simulink model "Vienna_Rectifier_PQ_Control"  (R2023b)
settings: Solver=VariableStepAuto  StartTime=0.0  StopTime=0.4  RelTol=1e-3
libraries: spsSeriesRLCBranchLib x6, spsIGBTLib x6, spsIGBTDiodeLib x6, spsVoltageMeasurementLib x5, spsCurrentMeasurementLib x3, spsRMSLib x3, spsACVoltageSourceLib x3, spsMeanLib x2, slpidlib x1, spsTHDLib x1, simulink x1, spspowerguiLib x1
settings Model: SimulationMode=accelerator  Creator=LXS  LastModifiedBy=Qu
settings SolverCC: ZeroCrossAlgorithm=Adaptive

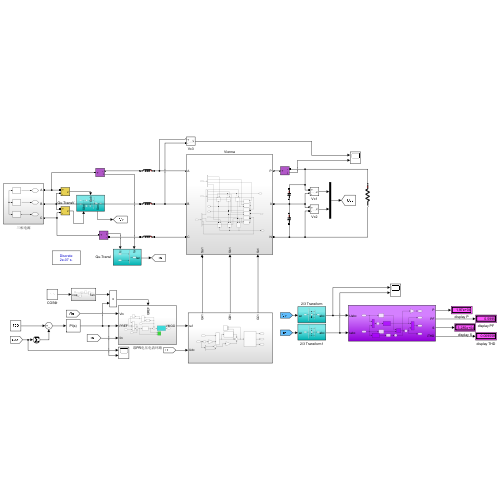
[thumbnail: Simulink's stored preview of the top-level diagram]
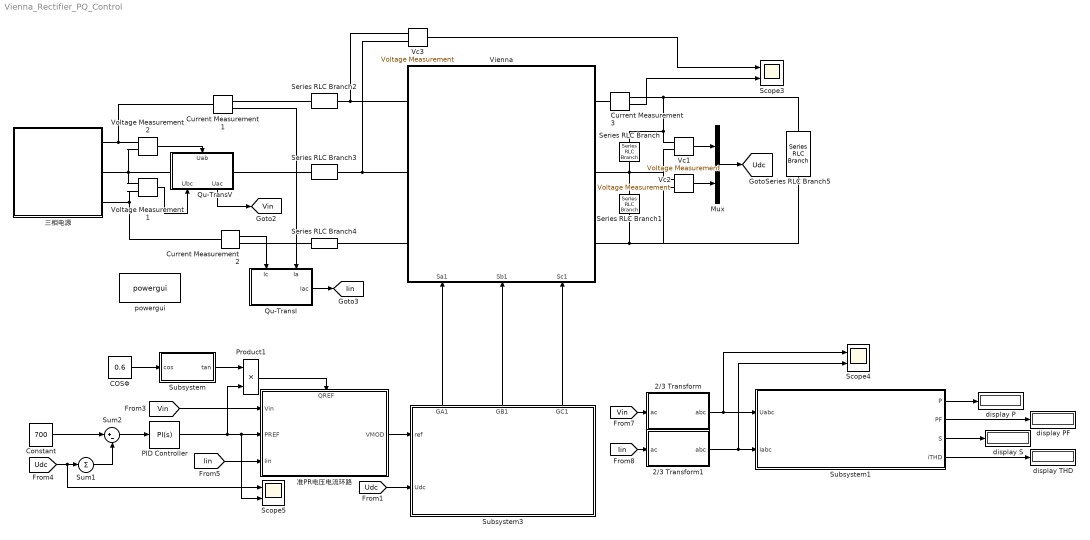
== system Vienna_Rectifier_PQ_Control ==
  2/3 Transform : Subsystem
      settings: PortSchema="{\"entries\":[{\"content\":{\"sides\":[{\"content\":{},\"type\":\"ConnectorPlacement.EquallySpacedRectSide\",\"uuid\":\"58c40194-9a95-4e39-952e-f878bde7484e\"},{\"content\":{\"side\":\"RIGHT\"},\"type\":\"ConnectorPlacement.EquallySpacedRectSide\",\"uuid\":\"f51692e8-3ff2-4d72-808d-3667196a4526\"},{\"content\":{\"connectorIds\":[\"In1\"],\"side\":\"TOP\"},\"type\":\"ConnectorPlacement.EquallySpacedRectSide\",\"uuid\":\"0aab136b-5da5-45c4-8998-999ebe8b7f2f\"},{\"content\":{\"connectorIds\":[\"Out1\"],\"side\":\"BOTTOM\"},\"type\":\"ConnectorPlacement.EquallySpacedRectSide\",\"uuid\":\"32f5f4a5-4ebb-496b-828d-b973bd46b44e\"}]},\"type\":\"ConnectorPlacement.EquallySpacedConnector\",\"uuid\":\"3ef81af7-d426-47fb-88e3-e33e58eebb83\"}],\"packageUris\":[\"http://schema.mathworks.com/mf0/Connector/R2020b\"],\"version\":\"1.0\"}"
  2/3 Transform1 : Subsystem
      settings: PortSchema="{\"entries\":[{\"content\":{\"sides\":[{\"content\":{},\"type\":\"ConnectorPlacement.EquallySpacedRectSide\",\"uuid\":\"58c40194-9a95-4e39-952e-f878bde7484e\"},{\"content\":{\"side\":\"RIGHT\"},\"type\":\"ConnectorPlacement.EquallySpacedRectSide\",\"uuid\":\"f51692e8-3ff2-4d72-808d-3667196a4526\"},{\"content\":{\"connectorIds\":[\"In1\"],\"side\":\"TOP\"},\"type\":\"ConnectorPlacement.EquallySpacedRectSide\",\"uuid\":\"0aab136b-5da5-45c4-8998-999ebe8b7f2f\"},{\"content\":{\"connectorIds\":[\"Out1\"],\"side\":\"BOTTOM\"},\"type\":\"ConnectorPlacement.EquallySpacedRectSide\",\"uuid\":\"32f5f4a5-4ebb-496b-828d-b973bd46b44e\"}]},\"type\":\"ConnectorPlacement.EquallySpacedConnector\",\"uuid\":\"3ef81af7-d426-47fb-88e3-e33e58eebb83\"}],\"packageUris\":[\"http://schema.mathworks.com/mf0/Connector/R2020b\"],\"version\":\"1.0\"}"
  COSΦ : Constant  Value=0.6
  Constant : Constant  Value=700
  Current Measurement1 : spsCurrentMeasurementLib/Current Measurement  PhasorSimulation=off  OutputType=Complex  PSBequivalent=0
  Current Measurement2 : spsCurrentMeasurementLib/Current Measurement  PhasorSimulation=off  OutputType=Complex  PSBequivalent=0
  Current Measurement3 : spsCurrentMeasurementLib/Current Measurement  PhasorSimulation=off  OutputType=Complex  PSBequivalent=0
  Mux : Mux  Inputs=2
  PID Controller : slpidlib/PID Controller  Controller=PI  Form=Parallel  TimeDomain=Continuous-time  UseExternalTs=off  SampleTime=-1  IntegratorMethod=Forward Euler  FilterMethod=Forward Euler  ControllerParametersSource=internal  P=0.15  I=10  UseKiTs=off  D=0  N=100  UseFilter=on  TunerSelectOption=Transfer Function Based (PID Tuner App)  InitialConditionSource=internal  InitialConditionForIntegrator=0  InitialConditionForFilter=0  DifferentiatorICPrevScaledInput=0  ExternalReset=none  TrackingMode=off  Kt=1  LimitOutput=off  SatLimitsSource=internal  UpperSaturationLimit=100  LowerSaturationLimit=-100  LinearizeAsGain=on  AntiWindupMode=none  Kb=1  LimitIntegrator=off  UpperIntegratorSaturationLimit=inf  LowerIntegratorSaturationLimit=-inf  POutMin=[]  POutMax=[]  IOutMin=[]  IOutMax=[]  DOutMin=[]  DOutMax=[]  NOutMin=[]  NOutMax=[]  SumOutMin=[]  SumOutMax=[]  SaturationOutMin=[]  SaturationOutMax=[]  PParamMin=[]  PParamMax=[]  IParamMin=[]  IParamMax=[]  DParamMin=[]  DParamMax=[]  NParamMin=[]  NParamMax=[]  KbParamMin=[]  KbParamMax=[]  KtParamMin=[]  KtParamMax=[]  KbOutMin=[]  KbOutMax=[]  KtOutMin=[]  KtOutMax=[]  IntegratorOutMin=[]  IntegratorOutMax=[]  FilterOutMin=[]  FilterOutMax=[]  SumI1OutMin=[]  SumI1OutMax=[]  SumI2OutMin=[]  SumI2OutMax=[]  SumI3OutMin=[]  SumI3OutMax=[]  SumI4OutMin=[]  SumI4OutMax=[]  SumDOutMin=[]  SumDOutMax=[]  DifferentiatorOutMin=[]  DifferentiatorOutMax=[]  FilterDiffOutCoefMin=[]  FilterDiffOutCoefMax=[]  ReciprocalOutMin=[]  ReciprocalOutMax=[]  SumDenOutMin=[]  SumDenOutMax=[]  SumNumOutMin=[]  SumNumOutMax=[]  DivideOutMin=[]  DivideOutMax=[]  UdiffTsProdOutMin=[]  UdiffTsProdOutMax=[]  NTsProdOutMin=[]  NTsProdOutMax=[]  UintegralTsProdOutMin=[]  UintegralTsProdOutMax=[]  UngainTsProdOutMin=[]  UngainTsProdOutMax=[]  ClampingZeroOutDataTypeStr=Inherit: Inherit via back propagation  ClampingZeroOutMin=[]  ClampingZeroOutMax=[]  FilterDenConstantOutDataTypeStr=Inherit: Inherit via back propagation  FilterDenConstantOutMin=[]  FilterDenConstantOutMax=[]  PCopyOutDataTypeStr=Inherit: Inherit via back propagation  PCopyOutMin=[]  PCopyOutMax=[]  NCopyOutDataTypeStr=Inherit: Inherit via back propagation  NCopyOutMin=[]  NCopyOutMax=[]  IntegratorContinuousStateAttributes=''  IntegratorStateMustResolveToSignalObject=off  IntegratorRTWStateStorageClass=Auto  FilterContinuousStateAttributes=''  FilterStateMustResolveToSignalObject=off  FilterRTWStateStorageClass=Auto  ParallelPVariant=InternalParameters  IdealPVariant=Disabled  IVariant=InternalParameters  DVariant=Disabled  IntegratorVariant=Continuous  SatVariant=Disabled  AWVariant=Passthrough  PCopyVariant=Disabled  TRVariant=Disabled  FdbkBlocksVariant=Forward  IdealPFdbkVariant=Disabled  SatFdbkVariant=Disabled  DerivativeFilterVariant=Disabled  NVariant=Disabled  NCopyVariant=Disabled_SignalSpec  FilterICVariant=Disabled  IntegratorICVariant=InternalICs  ExternalResetVariant=Disabled  TRSumVariant=Passthrough  SumFdbkVariant=Disabled  SumVariant=Sum_PI  TsampFilterVariant=InternalTs  TsampNgainVariant=Passthrough  TsampIntegralVariant=Disabled_SignalSpec  ExternalSaturationOutDataTypeStr=Inherit: Same as second input
  Product1 : Product
  Qu-TransI : Subsystem
      settings: PortSchema="{\"entries\":[{\"content\":{\"sides\":[{\"content\":{\"connectorIds\":[\"In1\",\"In2\"]},\"type\":\"ConnectorPlacement.EquallySpacedRectSide\",\"uuid\":\"58c40194-9a95-4e39-952e-f878bde7484e\"},{\"content\":{\"connectorIds\":[],\"side\":\"RIGHT\"},\"type\":\"ConnectorPlacement.EquallySpacedRectSide\",\"uuid\":\"f51692e8-3ff2-4d72-808d-3667196a4526\"},{\"content\":{\"connectorIds\":[],\"side\":\"TOP\"},\"type\":\"ConnectorPlacement.EquallySpacedRectSide\",\"uuid\":\"0aab136b-5da5-45c4-8998-999ebe8b7f2f\"},{\"content\":{\"connectorIds\":[\"Out1\"],\"side\":\"BOTTOM\"},\"type\":\"ConnectorPlacement.EquallySpacedRectSide\",\"uuid\":\"32f5f4a5-4ebb-496b-828d-b973bd46b44e\"}]},\"type\":\"ConnectorPlacement.EquallySpacedConnector\",\"uuid\":\"3ef81af7-d426-47fb-88e3-e33e58eebb83\"}],\"packageUris\":[\"http://schema.mathworks.com/mf0/Connector/R2020b\"],\"version\":\"1.0\"}"
  Qu-TransV : Subsystem
      settings: PortSchema="{\"entries\":[{\"content\":{\"sides\":[{\"content\":{\"connectorIds\":[\"In1\"]},\"type\":\"ConnectorPlacement.EquallySpacedRectSide\",\"uuid\":\"58c40194-9a95-4e39-952e-f878bde7484e\"},{\"content\":{\"connectorIds\":[\"In2\",\"Out1\"],\"side\":\"RIGHT\"},\"type\":\"ConnectorPlacement.EquallySpacedRectSide\",\"uuid\":\"f51692e8-3ff2-4d72-808d-3667196a4526\"},{\"content\":{\"side\":\"TOP\"},\"type\":\"ConnectorPlacement.EquallySpacedRectSide\",\"uuid\":\"0aab136b-5da5-45c4-8998-999ebe8b7f2f\"},{\"content\":{\"side\":\"BOTTOM\"},\"type\":\"ConnectorPlacement.EquallySpacedRectSide\",\"uuid\":\"185ce796-68e2-4136-8080-97dc86d2ba54\"}]},\"type\":\"ConnectorPlacement.EquallySpacedConnector\",\"uuid\":\"3ef81af7-d426-47fb-88e3-e33e58eebb83\"}],\"packageUris\":[\"http://schema.mathworks.com/mf0/Connector/R2020b\"],\"version\":\"1.0\"}"
  Scope3 : Scope  NumInputPorts=2
  Scope4 : Scope  NumInputPorts=2
  Scope5 : Scope  NumInputPorts=2
  Series RLC Branch : spsSeriesRLCBranchLib/Series RLC Branch  LConnTagsString=__new0  RConnTagsString=__new0  BranchType=C  Resistance=1  Inductance=1e-3  SetiL0=off  InitialCurrent=0  Capacitance=2e-3  Setx0=on  InitialVoltage=300  Measurements=None
  Series RLC Branch1 : spsSeriesRLCBranchLib/Series RLC Branch  LConnTagsString=__new0  RConnTagsString=__new0  BranchType=C  Resistance=1  Inductance=1e-3  SetiL0=off  InitialCurrent=0  Capacitance=2e-3  Setx0=on  InitialVoltage=300  Measurements=None
  Series RLC Branch2 : spsSeriesRLCBranchLib/Series RLC Branch  LConnTagsString=__new0  RConnTagsString=__new0  BranchType=L  Resistance=1  Inductance=5e-4  SetiL0=off  InitialCurrent=0  Capacitance=1e-6  Setx0=off  InitialVoltage=0  Measurements=None
  Series RLC Branch3 : spsSeriesRLCBranchLib/Series RLC Branch  LConnTagsString=__new0  RConnTagsString=__new0  BranchType=L  Resistance=1  Inductance=5e-4  SetiL0=off  InitialCurrent=0  Capacitance=1e-6  Setx0=off  InitialVoltage=0  Measurements=None
  Series RLC Branch4 : spsSeriesRLCBranchLib/Series RLC Branch  LConnTagsString=__new0  RConnTagsString=__new0  BranchType=L  Resistance=1  Inductance=5e-4  SetiL0=off  InitialCurrent=0  Capacitance=1e-6  Setx0=off  InitialVoltage=0  Measurements=None
  Series RLC Branch5 : spsSeriesRLCBranchLib/Series RLC Branch  LConnTagsString=__new0  RConnTagsString=__new0  BranchType=R  Resistance=25  Inductance=1e-3  SetiL0=off  InitialCurrent=0  Capacitance=1e-6  Setx0=off  InitialVoltage=0  Measurements=None
  Subsystem : Subsystem
  Subsystem1 : Subsystem
  Subsystem3 : Subsystem
      settings: PortSchema="{\"entries\":[{\"content\":{\"sides\":[{\"content\":{\"connectorIds\":[\"In1\",\"In2\"]},\"type\":\"ConnectorPlacement.EquallySpacedRectSide\",\"uuid\":\"86d8a801-af54-4615-919a-9a70996995f5\"},{\"content\":{\"side\":\"RIGHT\"},\"type\":\"ConnectorPlacement.EquallySpacedRectSide\",\"uuid\":\"9c099dd5-197a-4a29-8cd5-6822de601230\"},{\"content\":{\"connectorIds\":[\"Out1\",\"Out2\",\"Out3\"],\"side\":\"TOP\"},\"type\":\"ConnectorPlacement.EquallySpacedRectSide\",\"uuid\":\"5852d946-2383-4602-be71-32d16fa24bc3\"}]},\"type\":\"ConnectorPlacement.EquallySpacedConnector\",\"uuid\":\"a21c857f-e780-49b2-9a65-1676cf4540b1\"}],\"packageUris\":[\"http://schema.mathworks.com/mf0/Connector/R2020b\"],\"version\":\"1.0\"}"
  Sum1 : Sum  Inputs=+
  Sum2 : Sum  Inputs=|+-
  Vc1 : spsVoltageMeasurementLib/Voltage Measurement  PhasorSimulation=off  OutputType=Complex  PSBequivalent=0
  Vc2 : spsVoltageMeasurementLib/Voltage Measurement  PhasorSimulation=off  OutputType=Complex  PSBequivalent=0
  Vc3 : spsVoltageMeasurementLib/Voltage Measurement  PhasorSimulation=off  OutputType=Complex  PSBequivalent=0
  Vienna : Subsystem
      settings: PortSchema="{\"entries\":[{\"content\":{\"sides\":[{\"content\":{\"connectorIds\":[\"LConn1\",\"LConn2\",\"LConn3\"]},\"type\":\"ConnectorPlacement.EquallySpacedRectSide\",\"uuid\":\"b14efc91-6835-4ed7-8c1d-e2670cf7c179\"},{\"content\":{\"connectorIds\":[\"RConn1\",\"RConn2\",\"RConn3\"],\"side\":\"RIGHT\"},\"type\":\"ConnectorPlacement.EquallySpacedRectSide\",\"uuid\":\"133f26b8-b252-4d3c-80df-0b09760e0c14\"},{\"content\":{\"side\":\"TOP\"},\"type\":\"ConnectorPlacement.EquallySpacedRectSide\",\"uuid\":\"c058e102-7791-48c2-b9e4-e80cedcfd34e\"},{\"content\":{\"connectorIds\":[\"In1\",\"In2\",\"In3\"],\"side\":\"BOTTOM\"},\"type\":\"ConnectorPlacement.EquallySpacedRectSide\",\"uuid\":\"7bcd8845-3331-4b31-8039-611891643c20\"}]},\"type\":\"ConnectorPlacement.EquallySpacedConnector\",\"uuid\":\"173e4324-58a1-473c-9df3-d0606e4a673f\"}],\"packageUris\":[\"http://schema.mathworks.com/mf0/Connector/R2020b\"],\"version\":\"1.0\"}"
  Voltage Measurement1 : spsVoltageMeasurementLib/Voltage Measurement  PhasorSimulation=off  OutputType=Complex  PSBequivalent=0
  Voltage Measurement2 : spsVoltageMeasurementLib/Voltage Measurement  PhasorSimulation=off  OutputType=Complex  PSBequivalent=0
  display P : Display
  display PF : Display
  display S : Display
  display THD : Display
  powergui : spspowerguiLib/powergui  Priority=1  SimulationMode=Discrete  SampleTime=2e-7  frequency=60  Iterations=50  frequencyindice=50  Pbase=100e6  ErrMax=1e-4  UnitsV=kV  UnitsW=MW  buscounter=0  FunctionMessages=off  echomessages=off  EnableUseOfTLC=off  CurrentSourceSwitches=off  DisableSnubberDevices=off  DisableRonSwitches=off  DisableVfSwitches=off  DisplayEquations=off  AutomaticDiscreteSolvers=off  SolverType=Tustin/Backward Euler (TBE)  Interpol=off  ExternalGateDelay=off  methode=off  Ts=100  x0status=blocks  SPID=on  SwTol=0  HookPort=off  NonlinearTolerance=1e-4  nMaxIteration=100  ContinueOnMaxIteration=off  RestoreLinks=warning  ResistiveCurrentMeasurement=off  Frange=[0:2:500]  Ylog=off  Xlog=on  ShowGrid=off  save=off  variable=ZData  structure=0  ZoomFFT=off  StartTime=0.0  cycles=1  DisplayStyle=1  fundamental=60  FreqAxis=off  MaxFrequency=1000  frequencyindicesteady=1  RmsSteady=1  display=off
  三相电源 : Subsystem
  准PR电压电流环路 : Subsystem
      settings: PortSchema="{\"entries\":[{\"content\":{\"sides\":[{\"content\":{\"connectorIds\":[\"In1\",\"In2\",\"In3\"]},\"type\":\"ConnectorPlacement.EquallySpacedRectSide\",\"uuid\":\"dac3ff54-d1de-481a-901d-fe7d7474e460\"},{\"content\":{\"connectorIds\":[\"Out1\"],\"side\":\"RIGHT\"},\"type\":\"ConnectorPlacement.EquallySpacedRectSide\",\"uuid\":\"94b949b8-63b3-457c-8ea5-da44edec9bf3\"},{\"content\":{\"connectorIds\":[\"In4\"],\"side\":\"TOP\"},\"type\":\"ConnectorPlacement.EquallySpacedRectSide\",\"uuid\":\"1f5417c1-0a8c-48b6-bea3-1dc4e853aed2\"}]},\"type\":\"ConnectorPlacement.EquallySpacedConnector\",\"uuid\":\"5b0aae56-5e7d-4c0c-ad53-99d1136af505\"}],\"packageUris\":[\"http://schema.mathworks.com/mf0/Connector/R2020b\"],\"version\":\"1.0\"}"
  tag scope: Iin=global, Udc=global, Vin=global
  wires:
  Vc1/1 -> Mux/1
  Vc2/1 -> Mux/2
  Constant/1 -> Sum2/1
  Sum1/1 -> Sum2/2
  Sum2/1 -> PID Controller/1
  [Vin] -> 准PR电压电流环路/1(Vin)
  [Udc] -> Subsystem3/2(Udc)
  Subsystem1/3(S) -> display S/1
  Subsystem1/4(iTHD) -> display THD/1
  Subsystem1/2(PF) -> display PF/1
  Subsystem1/1(P) -> display P/1
  Subsystem3/3(GC1) -> Vienna/3(Sc1)
  Subsystem3/1(GA1) -> Vienna/1(Sa1)
  Subsystem3/2(GB1) -> Vienna/2(Sb1)
  [Udc] -> Scope5/1, Sum1/1
  Mux/1 -> [Udc]
  Vc3/1 -> Scope3/1
  Voltage Measurement2/1 -> Qu-TransV/1(Uab)
  Voltage Measurement1/1 -> Qu-TransV/2(Ubc)
  Qu-TransV/1(Uac) -> [Vin]
  Current Measurement2/1 -> Qu-TransI/1(Ic)
  Current Measurement1/1 -> Qu-TransI/2(Ia)
  Qu-TransI/1(Iac) -> [Iin]
  准PR电压电流环路/1(VMOD) -> Subsystem3/1(ref)
  PID Controller/1 -> Product1/2, Scope5/2, 准PR电压电流环路/2(PREF)
  [Iin] -> 准PR电压电流环路/3(Iin)
  2/3 Transform1/1(abc) -> Subsystem1/2(Iabc), Scope4/2
  2/3 Transform/1(abc) -> Subsystem1/1(Uabc), Scope4/1
  [Iin] -> 2/3 Transform1/1(ac)
  [Vin] -> 2/3 Transform/1(ac)
  Current Measurement3/1 -> Scope3/2
  Product1/1 -> 准PR电压电流环路/4(QREF)
  Subsystem/1(tan) -> Product1/1
  COSΦ/1 -> Subsystem/1(cos)
  connections:
  Series RLC Branch2/LConn1 -- Vienna/LConn1 -- Vc3/LConn1
  Series RLC Branch3/LConn1 -- Vc3/LConn2 -- Vienna/LConn2
  Series RLC Branch4/LConn1 -- Vienna/LConn3
  Series RLC Branch/RConn1 -- Vc1/LConn2 -- Vc2/LConn1 -- Series RLC Branch1/LConn1 -- Vienna/RConn2
  Series RLC Branch5/LConn1 -- Vc1/LConn1 -- Series RLC Branch/LConn1 -- Current Measurement3/RConn1
  三相电源/RConn1 -- Voltage Measurement2/LConn1 -- Current Measurement1/LConn1
  三相电源/RConn2 -- Voltage Measurement2/LConn2 -- Voltage Measurement1/LConn1 -- Series RLC Branch3/RConn1
  三相电源/RConn3 -- Current Measurement2/LConn1 -- Voltage Measurement1/LConn2
  Current Measurement1/RConn1 -- Series RLC Branch2/RConn1
  Current Measurement2/RConn1 -- Series RLC Branch4/RConn1
  Series RLC Branch1/RConn1 -- Series RLC Branch5/RConn1 -- Vc2/LConn2 -- Vienna/RConn3
  Current Measurement3/LConn1 -- Vienna/RConn1

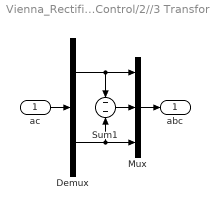
== system Vienna_Rectifier_PQ_Control/2//3 Transform ==
  ac : Inport
  Demux : Demux  Outputs=2
  Mux : Mux  Inputs=3
  Sum1 : Sum  Inputs=-|-
  abc : Outport
  wires:
  Sum1/1 -> Mux/2
  Mux/1 -> abc/1
  Demux/1 -> Sum1/1, Mux/1
  ac/1 -> Demux/1
  Demux/2 -> Sum1/2, Mux/3

== system Vienna_Rectifier_PQ_Control/2//3 Transform1 ==
  ac : Inport
  Demux : Demux  Outputs=2
  Mux : Mux  Inputs=3
  Sum1 : Sum  Inputs=-|-
  abc : Outport
  wires:
  Sum1/1 -> Mux/2
  Mux/1 -> abc/1
  Demux/1 -> Sum1/1, Mux/1
  ac/1 -> Demux/1
  Demux/2 -> Sum1/2, Mux/3

== system Vienna_Rectifier_PQ_Control/Qu-TransI ==
  Ic : Inport
  Ia : Inport  Port=2
  Mux : Mux  Inputs=2
  Iac : Outport
  wires:
  Ia/1 -> Mux/1
  Mux/1 -> Iac/1
  Ic/1 -> Mux/2

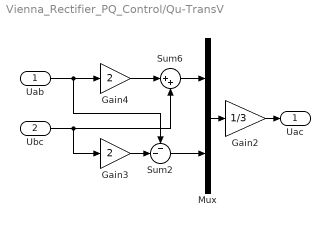
== system Vienna_Rectifier_PQ_Control/Qu-TransV ==
  Uab : Inport
  Ubc : Inport  Port=2
  Gain2 : Gain  Gain=1/3
  Gain3 : Gain  Gain=2
  Gain4 : Gain  Gain=2
  Mux : Mux  Inputs=2
  Sum2 : Sum  Inputs=--|
  Sum6 : Sum  Inputs=|++
  Uac : Outport
  wires:
  Uab/1 -> Sum2/1, Gain4/1
  Gain4/1 -> Sum6/1
  Ubc/1 -> Gain3/1, Sum6/2
  Sum2/1 -> Mux/2
  Sum6/1 -> Mux/1
  Gain3/1 -> Sum2/2
  Mux/1 -> Gain2/1
  Gain2/1 -> Uac/1

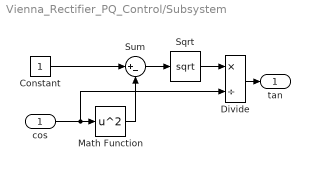
== system Vienna_Rectifier_PQ_Control/Subsystem ==
  cos : Inport
  Constant : Constant
  Divide : Product  Inputs=*/
  Math Function : Math  Operator=square
  Sqrt : Sqrt
  Sum : Sum  Inputs=|+-
  tan : Outport
  wires:
  cos/1 -> Divide/2, Math Function/1
  Math Function/1 -> Sum/2
  Constant/1 -> Sum/1
  Sum/1 -> Sqrt/1
  Sqrt/1 -> Divide/1
  Divide/1 -> tan/1

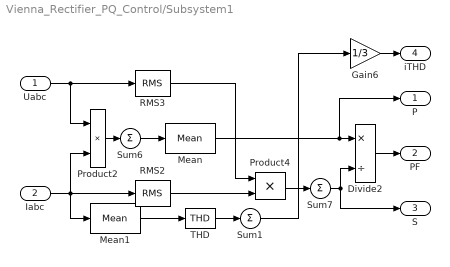
== system Vienna_Rectifier_PQ_Control/Subsystem1 ==
  Uabc : Inport
  Iabc : Inport  Port=2
  Divide2 : Product  Inputs=*/
  Gain6 : Gain  Gain=1/3
  Mean : spsMeanLib/Mean  Freq=100  Vinit=0  Ts=0
  Mean1 : spsMeanLib/Mean  Freq=20000  Vinit=0  Ts=0
  Product2 : Product
  Product4 : Product
  RMS2 : spsRMSLib/RMS  TrueRMS=on  Freq=50  RMSInit=0  Ts=0
  RMS3 : spsRMSLib/RMS  TrueRMS=on  Freq=50  RMSInit=0  Ts=0
  Sum1 : Sum  Inputs=+
  Sum6 : Sum  Inputs=+
  Sum7 : Sum  Inputs=+
  THD : spsTHDLib/THD  Freq=50  Ts=0
  P : Outport
  PF : Outport  Port=2
  S : Outport  Port=3
  iTHD : Outport  Port=4
  wires:
  Mean1/1 -> THD/1
  THD/1 -> Sum1/1
  Iabc/1 -> RMS2/1, Product2/2, Mean1/1
  Mean/1 -> Divide2/1, P/1
  Sum7/1 -> Divide2/2, S/1
  Uabc/1 -> Product2/1, RMS3/1
  Gain6/1 -> iTHD/1
  Sum1/1 -> Gain6/1
  RMS2/1 -> Product4/2
  Divide2/1 -> PF/1
  Product2/1 -> Sum6/1
  Sum6/1 -> Mean/1
  Product4/1 -> Sum7/1
  RMS3/1 -> Product4/1

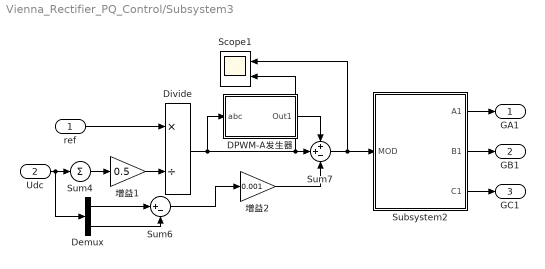
== system Vienna_Rectifier_PQ_Control/Subsystem3 ==
  ref : Inport
  Udc : Inport  Port=2
  DPWM-A发生器 : Subsystem
  Demux : Demux  Outputs=2
  Divide : Product  Inputs=*/
  Scope1 : Scope  NumInputPorts=2
  Subsystem2 : Subsystem
  Sum4 : Sum  Inputs=+
  Sum6 : Sum  Inputs=|+-
  Sum7 : Sum  Inputs=++-
  增益1 : Gain  Gain=0.5
  增益2 : Gain  Gain=0.001
  GA1 : Outport
  GB1 : Outport  Port=2
  GC1 : Outport  Port=3
  wires:
  Udc/1 -> Demux/1, Sum4/1
  ref/1 -> Divide/1
  Divide/1 -> Scope1/2, Sum7/2, DPWM-A发生器/1(abc)
  Sum7/1 -> Subsystem2/1(MOD), Scope1/1
  增益1/1 -> Divide/2
  Sum4/1 -> 增益1/1
  Subsystem2/3(C1) -> GC1/1
  Subsystem2/2(B1) -> GB1/1
  Subsystem2/1(A1) -> GA1/1
  DPWM-A发生器/1(Out1) -> Sum7/1
  Demux/1 -> Sum6/1
  Demux/2 -> Sum6/2
  Sum6/1 -> 增益2/1
  增益2/1 -> Sum7/3

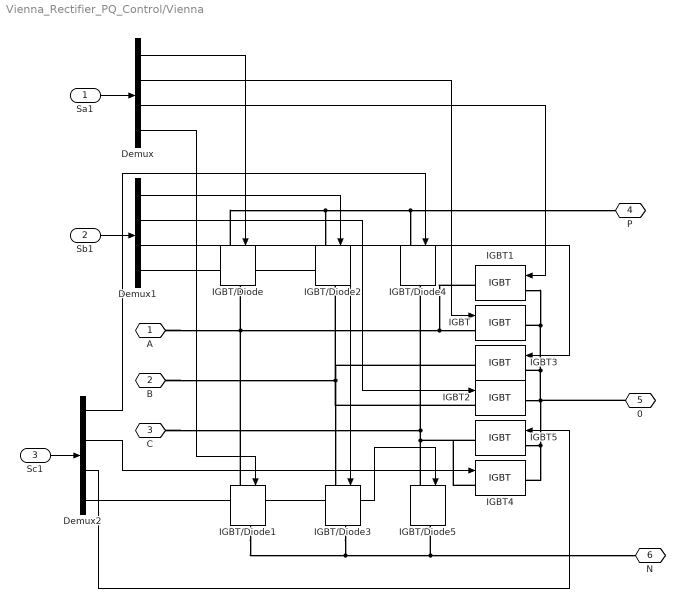
== system Vienna_Rectifier_PQ_Control/Vienna ==
  Sa1 : Inport
  Sb1 : Inport  Port=2
  Sc1 : Inport  Port=3
  Demux : Demux
  Demux1 : Demux
  Demux2 : Demux
  IGBT{,1..5} (6 alike) : spsIGBTLib/IGBT  Ron=0.001  Lon=0  Vf=1  Tf=1e-6  Tt=2e-6  IC=0  Rs=1e5  Cs=inf  Measurements=off
  IGBT/Diode{,1..5} (6 alike) : spsIGBTDiodeLib/IGBT//Diode  Ron=1e-3  Rs=1e5  Cs=inf  Measurements=off
  A : PMIOPort  Side=Left
  B : PMIOPort  Port=2  Side=Left
  C : PMIOPort  Port=3  Side=Left
  P : PMIOPort  Port=4  Side=Right
  0 : PMIOPort  Port=5  Side=Right
  N : PMIOPort  Port=6  Side=Right
  wires:
  Sa1/1 -> Demux/1
  Sb1/1 -> Demux1/1
  Sc1/1 -> Demux2/1
  Demux/2 -> IGBT/1
  Demux/3 -> IGBT1/1
  Demux/4 -> IGBT/Diode1/1
  Demux1/2 -> IGBT2/1
  Demux1/3 -> IGBT3/1
  Demux1/4 -> IGBT/Diode3/1
  Demux2/1 -> IGBT/Diode4/1
  Demux2/3 -> IGBT5/1
  Demux2/4 -> IGBT/Diode5/1
  Demux/1 -> IGBT/Diode/1
  Demux1/1 -> IGBT/Diode2/1
  Demux2/2 -> IGBT4/1
  connections:
  C/RConn1 -- IGBT4/LConn1 -- IGBT5/RConn1 -- IGBT/Diode5/LConn1 -- IGBT/Diode4/RConn1
  B/RConn1 -- IGBT2/LConn1 -- IGBT/Diode3/LConn1 -- IGBT/Diode2/RConn1 -- IGBT3/RConn1
  A/RConn1 -- IGBT/Diode/RConn1 -- IGBT1/RConn1 -- IGBT/LConn1 -- IGBT/Diode1/LConn1
  IGBT/Diode1/RConn1 -- IGBT/Diode3/RConn1 -- N/RConn1 -- IGBT/Diode5/RConn1
  IGBT/Diode/LConn1 -- IGBT/Diode2/LConn1 -- IGBT/Diode4/LConn1 -- P/RConn1
  IGBT2/RConn1 -- 0/RConn1 -- IGBT/RConn1 -- IGBT1/LConn1 -- IGBT3/LConn1 -- IGBT4/RConn1 -- IGBT5/LConn1

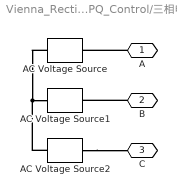
== system Vienna_Rectifier_PQ_Control/三相电源 ==
  AC Voltage Source : spsACVoltageSourceLib/AC Voltage Source  Amplitude=310  Phase=0  Frequency=50  SampleTime=0  Measurements=None  BusType=swing  Pref=10e3  Qref=0  Qmin=-inf  Qmax=+inf
  AC Voltage Source1 : spsACVoltageSourceLib/AC Voltage Source  Amplitude=310  Phase=120  Frequency=50  SampleTime=0  Measurements=None  BusType=swing  Pref=10e3  Qref=0  Qmin=-inf  Qmax=+inf
  AC Voltage Source2 : spsACVoltageSourceLib/AC Voltage Source  Amplitude=310  Phase=-120  Frequency=50  SampleTime=0  Measurements=None  BusType=swing  Pref=10e3  Qref=0  Qmin=-inf  Qmax=+inf
  A : PMIOPort  Side=Right
  B : PMIOPort  Port=2  Side=Right
  C : PMIOPort  Port=3  Side=Right
  connections:
  AC Voltage Source2/RConn1 -- C/RConn1
  A/RConn1 -- AC Voltage Source/RConn1
  B/RConn1 -- AC Voltage Source1/RConn1
  AC Voltage Source/LConn1 -- AC Voltage Source2/LConn1 -- AC Voltage Source1/LConn1

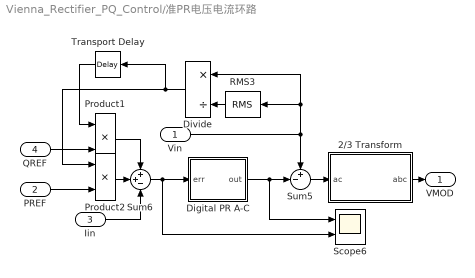
== system Vienna_Rectifier_PQ_Control/准PR电压电流环路 ==
  Vin : Inport
  PREF : Inport  Port=2
  Iin : Inport  Port=3
  QREF : Inport  Port=4
  2/3 Transform : Subsystem
      settings: PortSchema="{\"entries\":[{\"content\":{\"sides\":[{\"content\":{},\"type\":\"ConnectorPlacement.EquallySpacedRectSide\",\"uuid\":\"58c40194-9a95-4e39-952e-f878bde7484e\"},{\"content\":{\"side\":\"RIGHT\"},\"type\":\"ConnectorPlacement.EquallySpacedRectSide\",\"uuid\":\"f51692e8-3ff2-4d72-808d-3667196a4526\"},{\"content\":{\"connectorIds\":[\"In1\"],\"side\":\"TOP\"},\"type\":\"ConnectorPlacement.EquallySpacedRectSide\",\"uuid\":\"0aab136b-5da5-45c4-8998-999ebe8b7f2f\"},{\"content\":{\"connectorIds\":[\"Out1\"],\"side\":\"BOTTOM\"},\"type\":\"ConnectorPlacement.EquallySpacedRectSide\",\"uuid\":\"32f5f4a5-4ebb-496b-828d-b973bd46b44e\"}]},\"type\":\"ConnectorPlacement.EquallySpacedConnector\",\"uuid\":\"3ef81af7-d426-47fb-88e3-e33e58eebb83\"}],\"packageUris\":[\"http://schema.mathworks.com/mf0/Connector/R2020b\"],\"version\":\"1.0\"}"
  Digital PR A-C : Subsystem  mask{Kp=8, Kr=100, Wc=5, Ts=1/40000, Upper=600, Lower=-600}
      mask DialogControl ParameterGroupVar Prompt: 参数
  Divide : Product  Inputs=*/
  Product1 : Product
  Product2 : Product
  RMS3 : spsRMSLib/RMS  TrueRMS=on  Freq=50  RMSInit=220  Ts=0
  Scope6 : Scope  NumInputPorts=2
  Sum5 : Sum  Inputs=+-|
  Sum6 : Sum  Inputs=++-
  Transport Delay : TransportDelay  DelayTime=1/50/4
  VMOD : Outport
  wires:
  PREF/1 -> Product2/2
  Sum6/1 -> Digital PR A-C/1(err), Scope6/2
  Digital PR A-C/1(out) -> Scope6/1, Sum5/2
  Sum5/1 -> 2/3 Transform/1(ac)
  2/3 Transform/1(abc) -> VMOD/1
  Vin/1 -> Sum5/1, Divide/1, RMS3/1
  Iin/1 -> Sum6/3
  Product2/1 -> Sum6/2
  Product1/1 -> Sum6/1
  QREF/1 -> Product1/2
  RMS3/1 -> Divide/2
  Divide/1 -> Transport Delay/1, Product2/1
  Transport Delay/1 -> Product1/1

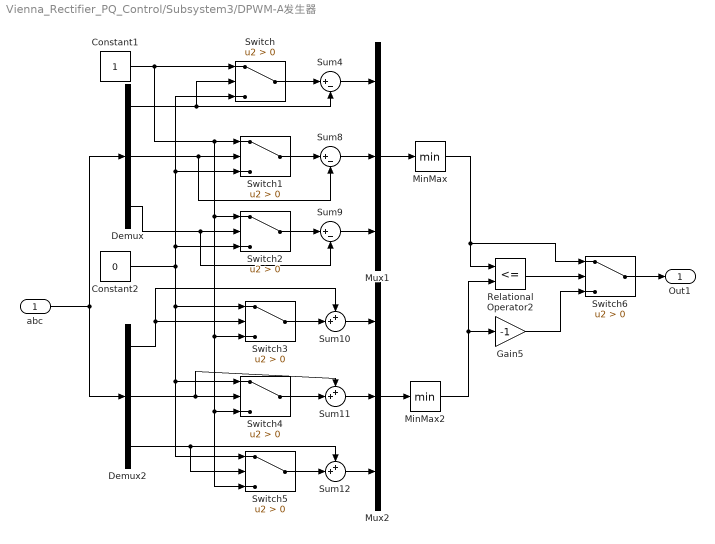
== system Vienna_Rectifier_PQ_Control/Subsystem3/DPWM-A发生器 ==
  abc : Inport
  Constant1 : Constant
  Constant2 : Constant  Value=0
  Demux : Demux  Outputs=3
  Demux2 : Demux  Outputs=3
  Gain5 : Gain  Gain=-1
  MinMax : MinMax
  MinMax2 : MinMax
  Mux1 : Mux  Inputs=3
  Mux2 : Mux  Inputs=3
  Relational Operator2 : RelationalOperator  Operator=<=  OutDataTypeStr=boolean  InputSameDT=off
  Sum10 : Sum  Inputs=++|
  Sum11 : Sum  Inputs=++|
  Sum12 : Sum  Inputs=++|
  Sum4 : Sum  Inputs=|+-
  Sum8 : Sum  Inputs=|+-
  Sum9 : Sum  Inputs=|+-
  Switch{,1..6} (7 alike) : Switch  Criteria=u2 > Threshold  SaturateOnIntegerOverflow=off  InputSameDT=off
  Out1 : Outport
  wires:
  Switch1/1 -> Sum8/1
  Constant1/1 -> Switch5/3, Switch4/3, Switch3/3, Switch2/1, Switch1/1, Switch/1
  Constant2/1 -> Switch1/3, Switch/3, Switch2/3, Switch5/1, Switch4/1, Switch3/1
  Demux2/2 -> Sum11/1, Switch4/2
  Sum9/1 -> Mux1/3
  Switch2/1 -> Sum9/1
  MinMax/1 -> Switch6/1, Relational Operator2/1
  Relational Operator2/1 -> Switch6/2
  Mux1/1 -> MinMax/1
  Mux2/1 -> MinMax2/1
  Sum10/1 -> Mux2/1
  Sum11/1 -> Mux2/2
  Switch/1 -> Sum4/1
  Demux/1 -> Sum4/2, Switch/2
  Demux2/1 -> Sum10/1, Switch3/2
  Demux/3 -> Sum9/2, Switch2/2
  Sum12/1 -> Mux2/3
  Gain5/1 -> Switch6/3
  Switch4/1 -> Sum11/2
  Demux/2 -> Sum8/2, Switch1/2
  MinMax2/1 -> Gain5/1, Relational Operator2/2
  Switch5/1 -> Sum12/2
  Demux2/3 -> Switch5/2, Sum12/1
  Sum8/1 -> Mux1/2
  Sum4/1 -> Mux1/1
  Switch3/1 -> Sum10/2
  abc/1 -> Demux/1, Demux2/1
  Switch6/1 -> Out1/1

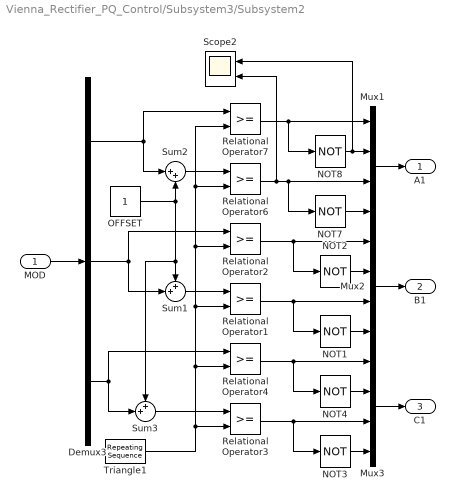
== system Vienna_Rectifier_PQ_Control/Subsystem3/Subsystem2 ==
  MOD : Inport
  Demux3 : Demux  Outputs=3
  Mux1 : Mux
  Mux2 : Mux
  Mux3 : Mux
  NOT{1..4,7..8} (6 alike) : Logic  Operator=NOT  IconShape=distinctive  AllPortsSameDT=off  OutDataTypeStr=boolean
  OFFSET : Constant
  Relational Operator{1..4,6..7} (6 alike) : RelationalOperator  OutDataTypeStr=boolean  InputSameDT=off
  Scope2 : Scope  NumInputPorts=2
  Sum1 : Sum  Inputs=++|
  Sum2 : Sum  Inputs=|++
  Sum3 : Sum  Inputs=++|
  Triangle1 : simulink/Sources/Repeating Sequence  rep_seq_t=[0 1/20000/2 1/20000]  rep_seq_y=[0 1 0]
  A1 : Outport
  B1 : Outport  Port=2
  C1 : Outport  Port=3
  wires:
  MOD/1 -> Demux3/1
  Mux1/1 -> A1/1
  Mux3/1 -> C1/1
  Mux2/1 -> B1/1
  OFFSET/1 -> Sum3/1, Sum1/1, Sum2/2
  Relational Operator6/1 -> Scope2/2, NOT7/1, Mux1/3
  Sum2/1 -> Relational Operator6/1
  NOT7/1 -> Mux1/4
  Relational Operator7/1 -> Mux1/1, NOT8/1
  Triangle1/1 -> Relational Operator3/2, Relational Operator4/2, Relational Operator1/2, Relational Operator2/2, Relational Operator7/2, Relational Operator6/2
  NOT8/1 -> Scope2/1, Mux1/2
  Demux3/1 -> Sum2/1, Relational Operator7/1
  Relational Operator2/1 -> Mux2/1, NOT2/1
  Relational Operator1/1 -> NOT1/1, Mux2/3
  NOT2/1 -> Mux2/2
  NOT1/1 -> Mux2/4
  NOT3/1 -> Mux3/4
  NOT4/1 -> Mux3/2
  Relational Operator3/1 -> Mux3/3, NOT3/1
  Relational Operator4/1 -> Mux3/1, NOT4/1
  Demux3/2 -> Relational Operator2/1, Sum1/2
  Sum1/1 -> Relational Operator1/1
  Sum3/1 -> Relational Operator3/1
  Demux3/3 -> Relational Operator4/1, Sum3/2

== system Vienna_Rectifier_PQ_Control/准PR电压电流环路/2//3 Transform ==
  ac : Inport
  Demux : Demux  Outputs=2
  Mux : Mux  Inputs=3
  Sum1 : Sum  Inputs=-|-
  abc : Outport
  wires:
  Sum1/1 -> Mux/2
  Mux/1 -> abc/1
  Demux/1 -> Sum1/1, Mux/1
  ac/1 -> Demux/1
  Demux/2 -> Sum1/2, Mux/3

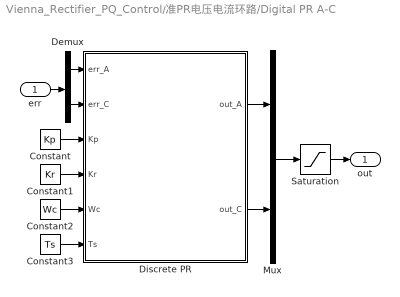
== system Vienna_Rectifier_PQ_Control/准PR电压电流环路/Digital PR A-C ==
  err : Inport
  Constant : Constant  Value=Kp
  Constant1 : Constant  Value=Kr
  Constant2 : Constant  Value=Wc
  Constant3 : Constant  Value=Ts
  Demux : Demux  Outputs=2
  Discrete PR : MATLAB Function  TreatAsAtomicUnit=on
  Mux : Mux  Inputs=2
  Saturation : Saturate  UpperLimit=Upper  LowerLimit=Lower
  out : Outport
  wires:
  Constant1/1 -> Discrete PR/4(Kr)
  Constant3/1 -> Discrete PR/6(Ts)
  Constant/1 -> Discrete PR/3(Kp)
  Constant2/1 -> Discrete PR/5(Wc)
  Demux/1 -> Discrete PR/1(err_A)
  err/1 -> Demux/1
  Demux/2 -> Discrete PR/2(err_C)
  Discrete PR/1(out_A) -> Mux/1
  Discrete PR/2(out_C) -> Mux/2
  Mux/1 -> Saturation/1
  Saturation/1 -> out/1

== matlab function Vienna_Rectifier_PQ_Control/准PR电压电流环路/Digital PR A-C/Discrete PR ==
  settings: updateMethod=DISCRETE  sampleTime=Ts
  data: err_A input; err_C input; out_A output; Kp input; Kr input; Wc input; Ts input; out_C output
function [out_A, out_C] = fcn(err_A, err_C, Kp, Kr, Wc, Ts)

W0 = 50*2*pi;

%%定义三相静态变量
persistent err_A1;
persistent err_A2;
persistent out_A1;
persistent out_A2;

persistent err_C1;
persistent err_C2;
persistent out_C1;
persistent out_C2;

%%对三相静态变量初始化
if isempty(err_A1)
    err_A1 = 0;
end
if isempty(err_A2)
    err_A2 = 0;
end
if isempty(out_A1)
    out_A1 = 0;
end
if isempty(out_A2)
    out_A2 = 0;
end


if isempty(err_C1)
    err_C1 = 0;
end
if isempty(err_C2)
    err_C2 = 0;
end
if isempty(out_C1)
    out_C1 = 0;
end
if isempty(out_C2)
    out_C2 = 0;
end

%%Discrete
t1 = Wc * Ts;
t2 = W0^2 * Ts^2;
t3 = t2 + 4*t1 + 4;

b0 = (Kp*t2 + 4*(Kp+Kr)*t1 + 4*Kp) / t3;
b1 = (2*Kp*t2 - 8*Kp) / t3;
b2 = (Kp*t2 + 4*Kp - 4*(Kp+Kr)*t1) / t3;
a1 = (2*t2 - 8) / t3;
a2 = (t2 - 4*t1 + 4) / t3;

%%计算三相输出量
out_A = b0*err_A + b1*err_A1 + b2*err_A2 - a1*out_A1 - a2*out_A2;
out_A2 = out_A1;
out_A1 = out_A;
err_A2 = err_A1;
err_A1 = err_A;


out_C = b0*err_C + b1*err_C1 + b2*err_C2 - a1*out_C1 - a2*out_C2;
out_C2 = out_C1;
out_C1 = out_C;
err_C2 = err_C1;
err_C1 = err_C;
